simulink model "INVERTER_CTRL"  (R2023a)
settings: Solver=FixedStepAuto  StartTime=0.0  StopTime=Inf  FixedStep=1e-5  RelTol=1e-3  EnableMultiTasking=on
undefined symbols (not defined in the file or in its folder): DiscIntNeverNeededParam
libraries: c2837xDlib x4, c2802xlib x3, simulink x1, spspowerguiLib x1
settings Model: ExtModeTrigDuration=8  Creator=RAGHAVA  LastModifiedBy=RAGHAVA
settings SolverCC: AutoInsertRateTranBlk=on
settings OptimizationCC: DefaultUnderspecifiedDataType=single  EnhancedBackFolding=on  PassReuseOutputArgsAs=Individual arguments  MaxStackSize=1024  OptimizeBlockOrder=speed  DifferentSizesBufferReuse=on  OptimizationCustomize=off  DenormalBehavior=FlushToZero  EfficientTunableParamExpr=on
settings DebuggingCC: ParameterTunabilityLossMsg=error
settings HardwareCC: ProdBitPerChar=16  ProdBitPerInt=16  ProdBitPerPointer=32  ProdBitPerSizeT=32  ProdBitPerPtrDiffT=32  ProdLargestAtomicInteger=Integer  ProdLargestAtomicFloat=None  ProdWordSize=16  ProdLongLongMode=on  ProdHWDeviceType=Texas Instruments->C2000  HardwareBoardFeatureSet=SoCBlockset
settings ModelReferenceCC: ModelReferenceNumInstancesAllowed=Single
settings SFSimCC: MATLABDynamicMemAlloc=off
settings RTWCC: Description=Embedded Coder  SystemTargetFile=ert.tlc  HardwareBoard=TI Delfino F28379D LaunchPad  TemplateMakefile=ert_default_tmf  Toolchain=Texas Instruments Code Composer Studio (C2000)
settings CodeAppCC: ForceParamTrailComments=on  IgnoreCustomStorageClasses=off  OperatorAnnotations=on  SimulinkDataObjDesc=on  SFDataObjDesc=on  InsertBlockDesc=on
settings ERTTargetCC: CodeReplacementLibrary=TI C28x  SupportContinuousTime=on  ExtModeTransport=4  ExtModeStaticAlloc=on  ExtModeAutomaticAllocSize=off  ExtModeStaticAllocSize=10000  ExtModeMexFile=ext_xcp  ExtModeIntrfLevel=Level2 - Open

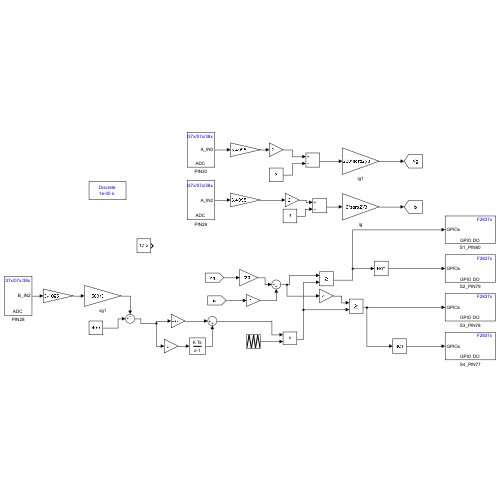
[thumbnail: Simulink's stored preview of the top-level diagram]
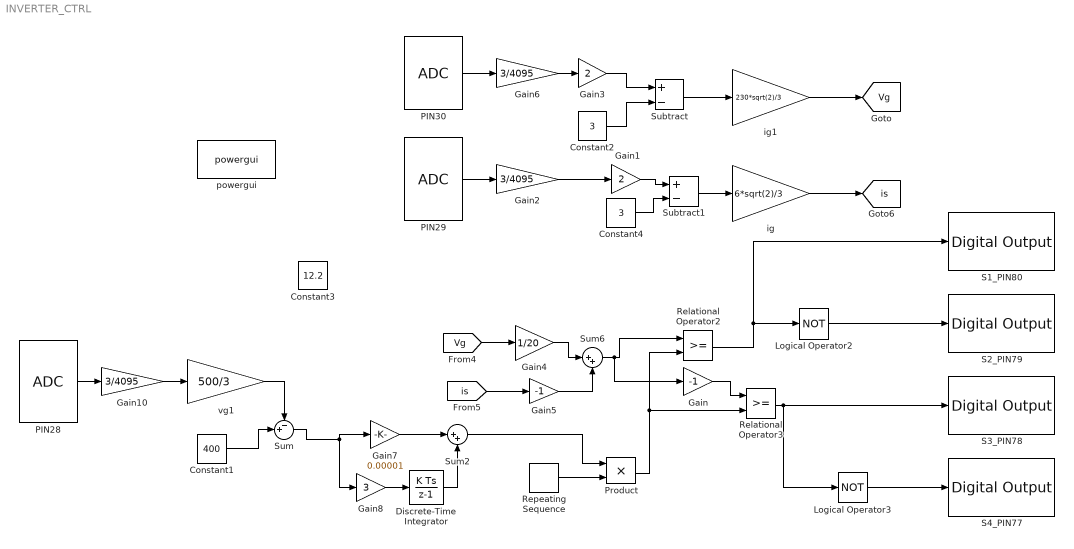
== system INVERTER_CTRL ==
  Constant1 : Constant  Value=400
  Constant2 : Constant  Value=3
  Constant3 : Constant  Value=12.2
  Constant4 : Constant  Value=3
  Discrete-Time Integrator : DiscreteIntegrator  SampleTime=1e-5  ICPrevOutput=DiscIntNeverNeededParam  ICPrevScaledInput=DiscIntNeverNeededParam
  Gain : Gain  Gain=-1
  Gain1 : Gain  Gain=2
  Gain10 : Gain  Gain=3/4095
  Gain2 : Gain  Gain=3/4095
  Gain3 : Gain  Gain=2
  Gain4 : Gain  Gain=1/20
  Gain5 : Gain  Gain=-1
  Gain6 : Gain  Gain=3/4095
  Gain7 : Gain  Gain=0.00001
  Gain8 : Gain  Gain=3
  Logical Operator2 : Logic  Operator=NOT  AllPortsSameDT=off  OutDataTypeStr=boolean
  Logical Operator3 : Logic  Operator=NOT  AllPortsSameDT=off  OutDataTypeStr=boolean
  PIN28 : c2802xlib/ADC  blkParamProc=C2000_Type4  ADCModule=B  samplingMode=Single sample mode  ADCResolution=12-bit (Single-ended input)  useSOC1=SOC2  useSOC2=SOC0_SOC1  SOCAcquisitionWindow=15  SOCTriggerSource=Software  SOCInterruptTrigger=No ADCINT  Ts=1e-5  dType=double  postInterrupt=off  interruptSel=ADCINT1  ADCINTContinuous=on  endma=off  chdma=1  conv1=ADCINA0  conv2=ADCINA0 and ADCINB0  conv1_Type4=ADCIN2  conv2_Type4=ADCIN0 and ADCIN1
      settings: LibrarySourceBlock=c2837xDlib/ADC
  PIN29 : c2802xlib/ADC  blkParamProc=C2000_Type4  ADCModule=A  samplingMode=Single sample mode  ADCResolution=12-bit (Single-ended input)  useSOC1=SOC2  useSOC2=SOC0_SOC1  SOCAcquisitionWindow=15  SOCTriggerSource=Software  SOCInterruptTrigger=No ADCINT  Ts=1e-5  dType=double  postInterrupt=off  interruptSel=ADCINT1  ADCINTContinuous=on  endma=off  chdma=1  conv1=ADCINA0  conv2=ADCINA0 and ADCINB0  conv1_Type4=ADCIN2  conv2_Type4=ADCIN0 and ADCIN1
      settings: LibrarySourceBlock=c2837xDlib/ADC
  PIN30 : c2802xlib/ADC  blkParamProc=C2000_Type4  ADCModule=A  samplingMode=Single sample mode  ADCResolution=12-bit (Single-ended input)  useSOC1=SOC0  useSOC2=SOC0_SOC1  SOCAcquisitionWindow=15  SOCTriggerSource=Software  SOCInterruptTrigger=No ADCINT  Ts=1e-5  dType=double  postInterrupt=off  interruptSel=ADCINT1  ADCINTContinuous=on  endma=off  chdma=1  conv1=ADCINA0  conv2=ADCINA0 and ADCINB0  conv1_Type4=ADCIN0  conv2_Type4=ADCIN0 and ADCIN1
      settings: LibrarySourceBlock=c2837xDlib/ADC
  Product : Product
  Relational Operator2 : RelationalOperator  OutDataTypeStr=boolean  RndMeth=Simplest  InputSameDT=off
  Relational Operator3 : RelationalOperator  OutDataTypeStr=boolean  RndMeth=Simplest  InputSameDT=off
  Repeating Sequence : simulink/Sources/Repeating Sequence  rep_seq_t=[0 0.5 1]*(1/10000)  rep_seq_y=[-1 1 -1]
  S1_PIN80 : c2837xDlib/Digital Output  GPIO_Number=GPIO0~GPIO7  GPIO_Bit0=off  GPIO_BIT0_Toggle=off  GPIO_Bit1=off  GPIO_BIT1_Toggle=off  GPIO_Bit2=off  GPIO_BIT2_Toggle=off  GPIO_Bit3=off  GPIO_BIT3_Toggle=off  GPIO_Bit4=off  GPIO_BIT4_Toggle=off  GPIO_Bit5=off  GPIO_BIT5_Toggle=off  GPIO_Bit6=on  GPIO_BIT6_Toggle=off  GPIO_Bit7=off  GPIO_BIT7_Toggle=off
  S2_PIN79 : c2837xDlib/Digital Output  GPIO_Number=GPIO0~GPIO7  GPIO_Bit0=off  GPIO_BIT0_Toggle=off  GPIO_Bit1=off  GPIO_BIT1_Toggle=off  GPIO_Bit2=off  GPIO_BIT2_Toggle=off  GPIO_Bit3=off  GPIO_BIT3_Toggle=off  GPIO_Bit4=off  GPIO_BIT4_Toggle=off  GPIO_Bit5=off  GPIO_BIT5_Toggle=off  GPIO_Bit6=off  GPIO_BIT6_Toggle=off  GPIO_Bit7=on  GPIO_BIT7_Toggle=off
  S3_PIN78 : c2837xDlib/Digital Output  GPIO_Number=GPIO8~GPIO15  GPIO_Bit0=on  GPIO_BIT0_Toggle=off  GPIO_Bit1=off  GPIO_BIT1_Toggle=off  GPIO_Bit2=off  GPIO_BIT2_Toggle=off  GPIO_Bit3=off  GPIO_BIT3_Toggle=off  GPIO_Bit4=off  GPIO_BIT4_Toggle=off  GPIO_Bit5=off  GPIO_BIT5_Toggle=off  GPIO_Bit6=off  GPIO_BIT6_Toggle=off  GPIO_Bit7=off  GPIO_BIT7_Toggle=off
  S4_PIN77 : c2837xDlib/Digital Output  GPIO_Number=GPIO8~GPIO15  GPIO_Bit0=off  GPIO_BIT0_Toggle=off  GPIO_Bit1=on  GPIO_BIT1_Toggle=off  GPIO_Bit2=off  GPIO_BIT2_Toggle=off  GPIO_Bit3=off  GPIO_BIT3_Toggle=off  GPIO_Bit4=off  GPIO_BIT4_Toggle=off  GPIO_Bit5=off  GPIO_BIT5_Toggle=off  GPIO_Bit6=off  GPIO_BIT6_Toggle=off  GPIO_Bit7=off  GPIO_BIT7_Toggle=off
  Subtract : Sum  Inputs=+-
  Subtract1 : Sum  Inputs=+-
  Sum : Sum  Inputs=-+|
  Sum2 : Sum  Inputs=|++
  Sum6 : Sum  Inputs=|++
  ig : Gain  Gain=6*sqrt(2)/3
  ig1 : Gain  Gain=230*sqrt(2)/3
  powergui : spspowerguiLib/powergui  Priority=1  SimulationMode=Discrete  SampleTime=1e-5  frequency=60  Iterations=50  frequencyindice=60  Pbase=100e6  ErrMax=1e-4  UnitsV=kV  UnitsW=MW  buscounter=0  FunctionMessages=off  echomessages=off  EnableUseOfTLC=off  CurrentSourceSwitches=off  DisableSnubberDevices=off  DisableRonSwitches=off  DisableVfSwitches=off  DisplayEquations=off  AutomaticDiscreteSolvers=off  SolverType=Tustin/Backward Euler (TBE)  Interpol=off  ExternalGateDelay=off  methode=off  Ts=100  x0status=blocks  SPID=on  SwTol=0  HookPort=off  NonlinearTolerance=1e-4  nMaxIteration=100  ContinueOnMaxIteration=off  RestoreLinks=warning  ResistiveCurrentMeasurement=off  Frange=[0:2:500]  Ylog=off  Xlog=on  ShowGrid=off  save=off  variable=ZData  structure=0  ZoomFFT=off  StartTime=0.0  cycles=1  DisplayStyle=1  fundamental=60  FreqAxis=off  MaxFrequency=1000  frequencyindicesteady=1  RmsSteady=1  display=off
  vg1 : Gain  Gain=500/3
  tag scope: Vg=global, is=global
  wires:
  Subtract/1 -> ig1/1
  Constant2/1 -> Subtract/2
  Gain3/1 -> Subtract/1
  Gain5/1 -> Sum6/2
  Logical Operator3/1 -> S4_PIN77/1
  Sum6/1 -> Gain/1, Relational Operator2/1
  Relational Operator3/1 -> Logical Operator3/1, S3_PIN78/1
  [is] -> Gain5/1
  Relational Operator2/1 -> S1_PIN80/1, Logical Operator2/1
  Repeating Sequence/1 -> Product/2
  [Vg] -> Gain4/1
  Logical Operator2/1 -> S2_PIN79/1
  Product/1 -> Relational Operator2/2, Relational Operator3/2
  Gain4/1 -> Sum6/1
  Gain/1 -> Relational Operator3/1
  ig1/1 -> [Vg]
  ig/1 -> [is]
  Gain1/1 -> Subtract1/1
  Constant4/1 -> Subtract1/2
  Subtract1/1 -> ig/1
  Gain2/1 -> Gain1/1
  Gain6/1 -> Gain3/1
  PIN30/1 -> Gain6/1
  PIN29/1 -> Gain2/1
  Gain7/1 -> Sum2/1
  Sum/1 -> Gain7/1, Gain8/1
  Constant1/1 -> Sum/2
  Discrete-Time Integrator/1 -> Sum2/2
  Gain8/1 -> Discrete-Time Integrator/1
  PIN28/1 -> Gain10/1
  Gain10/1 -> vg1/1
  vg1/1 -> Sum/1
  Sum2/1 -> Product/1
